simulink model "AlphaBotKreisfahrt"  (R2026b)
settings: Solver=FixedStepDiscrete  StopTime=inf  FixedStep=PAR_Sys_AbtastBasis_f64  EnableMultiTasking=on
StopFcn:
  | SpeichereKreisfahrt('AlphaBotKreisfahrt');
model workspace (MAT data in the model file):
  PAR_AktMot_PWM0_u8 = 80
  PAR_AktMot_RichtL_u8 = 0
  PAR_AktMot_RichtR_u8 = 0
  PAR_AktMot_Start_f32 = Simulink.Parameter
  PAR_AktMot_Start_f32.Value = 0
  PAR_AktMot_Start_f32.Complexity = 'real'
  PAR_AktMot_Start_f32.Dimensions = [1 1]
  PAR_AktMot_Start_f32.DataType = 'single'
  PAR_RegKrs_Ki_f32 = 2
  PAR_RegKrs_Kp_f32 = 0.20000000298
  PAR_RegKrs_RSoll_f32 = 1
  PAR_RegKrs_TKreis_f64 = 40
  PAR_RegKrs_VSoll_f32 = 0.34999999404
  PAR_SenGyr_NKalib_f64 = 1000
  PAR_SenGyr_Vorz_f32 = 1
  PAR_SenOdo_IncU_f32 = 40
  PAR_SenOdo_KorrSL_f32 = 1
  PAR_SenOdo_RadR_f32 = 0.0320000015199
  PAR_SenOdo_Spur_f32 = 0.140000000596
  PAR_Sys_AbtastBasis_f64 = 0.01
  PAR_Sys_Abtast_f64 = 0.01
libraries: arduinolib x8, arduinosensorlib x1
settings Model: SILPILModeSetting=veronly  SimulationMode=external
settings SolverCC: AutoInsertRateTranBlk=on
settings OptimizationCC: DifferentSizesBufferReuse=on  EfficientTunableParamExpr=on  EnhancedBackFolding=on  MaxStackSize=64  OptimizationCustomize=off  OptimizeBlockOrder=speed  PassReuseOutputArgsAs=Individual arguments  RemoveInternalMemoryZeroInit=on  RemoveRootLevelIOMemoryZeroInit=on
settings DebuggingCC: ParameterTunabilityLossMsg=error
settings HardwareCC: ProdHWDeviceType=ARM Compatible->ARM Cortex  ProdLargestAtomicFloat=Double  ProdLargestAtomicInteger=Long
settings SFSimCC: MATLABDynamicMemAlloc=off
settings RTWCC: BuildConfiguration=Faster Runs  Description=Embedded Coder  HardwareBoard=Arduino Uno R4 WiFi  SystemTargetFile=ert.tlc  TLCOptions=-aInlineSetEventsForThisBaseRateFcn=TLC_FALSE -aSuppressMultiTaskScheduler=TLC_FALSE -aRateBasedStepFcn=1  TemplateMakefile=ert_default_tmf  Toolchain=Arduino ARM M4
settings CodeAppCC: ForceParamTrailComments=on  IgnoreCustomStorageClasses=off  InsertBlockDesc=on  OperatorAnnotations=on  SFDataObjDesc=on  SimulinkDataObjDesc=on
settings ERTTargetCC: CombineSignalStateStructs=on  ExtModeAutomaticAllocSize=off  ExtModeIntrfLevel=Level2 - Open  ExtModeMexFile=ext_xcp  ExtModeStaticAlloc=on  SupportContinuousTime=on  SupportVariableSizeSignals=on

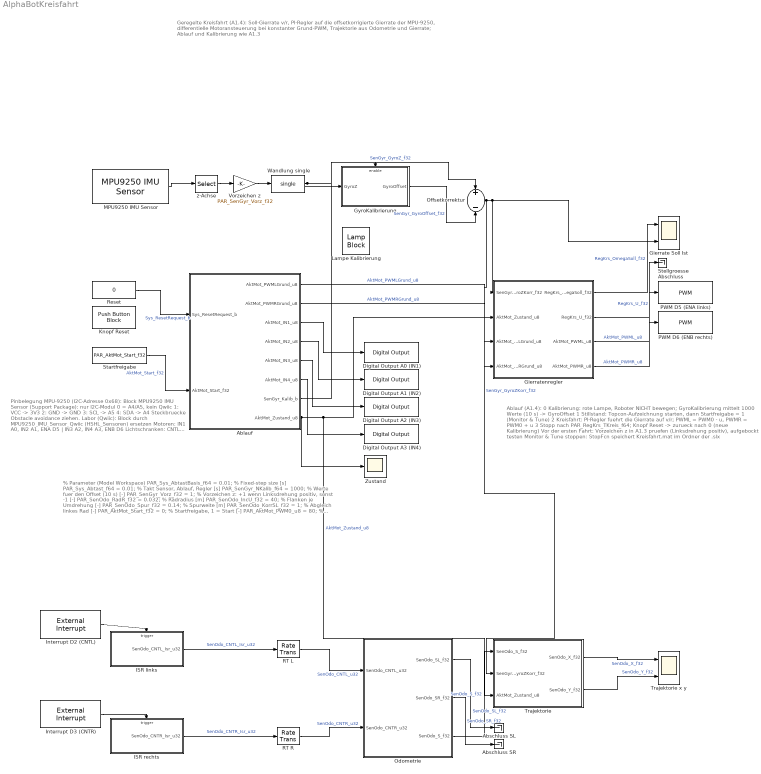
== system AlphaBotKreisfahrt ==
  note: % Parameter (Model Workspace)
      | PAR_Sys_AbtastBasis_f64 = 0.01; % Fixed-step size [s]
      | PAR_Sys_Abtast_f64 = 0.01; % Takt Sensor, Ablauf, Regler [s]
      | PAR_SenGyr_NKalib_f64 = 1000; % Werte fuer den Offset (10 s) [-]
      | PAR_SenGyr_Vorz_f32 = 1; % Vorzeichen z: +1 wenn Linksdrehung positiv, sonst -1 [-]
      | PAR_SenOdo_RadR_f32 = 0.032; % Radradius [m]
      | PAR_SenOdo_IncU_f32 = 40; % Flanken je Umdrehung [-]
      | PAR_SenOdo_Spur_f32 = 0.14; % Spurweite [m]
      | PAR_SenOdo_KorrSL_f32 = 1; % Abgleich linkes Rad [-]
      | PAR_AktMot_Start_f32 = 0; % Startfreigabe, 1 = Start [-]
      | PAR_AktMot_PWM0_u8 = 80; % Grund-PWM, mittlere Geschwindigkeit [-]
      | PAR_AktMot_RichtL_u8 = 0; % IN1 vorwaerts links, IN2 = 1 - IN1 [-]
      | PAR_AktMot_RichtR_u8 = 1; % IN3 vorwaerts rechts, IN4 = 1 - IN3 [-]
      | PAR_RegKrs_VSoll_f32 = 0.35; % Sollgeschwindigkeit [m/s]
      | PAR_RegKrs_RSoll_f32 = 1.0; % Sollradius [m]
      | PAR_RegKrs_Kp_f32 = 0.2; % PI: Verstaerkung [1/(Grad/s)]
      | PAR_RegKrs_Ki_f32 = 2.0; % PI: Integralverstaerkung [1/Grad]
      | PAR_RegKrs_TKreis_f64 = 40; % Dauer Kreisfahrt [s]
  note: Geregelte Kreisfahrt (A1.4): Soll-Gierrate v/r, PI-Regler auf die offsetkorrigierte Gierrate der MPU-9250, differentielle Motoransteuerung bei konstanter Grund-PWM, Trajektorie aus Odometrie und Gierrate; Ablauf und Kalibrierung wie A1.3
  note: Pinbelegung MPU-9250 (I2C-Adresse 0x68):
      | Block MPU9250 IMU Sensor (Support Package): nur I2C-Modul 0 = A4/A5, kein Qwiic
      | 1: VCC -> 3V3 2: GND -> GND 3: SCL -> A5 4: SDA -> A4
      | Steckbruecke Obstacle avoidance ziehen. Labor (Qwiic): Block durch MPU9250_IMU_Sensor_Qwiic (HSHL_Sensoren) ersetzen
      | Motoren: IN1 A0, IN2 A1, ENA D5 | IN3 A2, IN4 A3, ENB D6
      | Lichtschranken: CNTL D2, CNTR D3 (Interrupt, CHANGE)
  note: Ablauf (A1.4):
      | 0 Kalibrierung: rote Lampe, Roboter NICHT bewegen; GyroKalibrierung mittelt 1000 Werte (10 s) -> GyroOffset
      | 1 Stillstand: Topcon-Aufzeichnung starten, dann Startfreigabe = 1 (Monitor & Tune)
      | 2 Kreisfahrt: PI-Regler fuehrt die Gierrate auf v/r; PWML = PWM0 - u, PWMR = PWM0 + u
      | 3 Stopp nach PAR_RegKrs_TKreis_f64; Knopf Reset -> zurueck nach 0 (neue Kalibrierung)
      | Vor der ersten Fahrt: Vorzeichen z in A1.3 pruefen (Linksdrehung positiv), aufgebockt testen
      | Monitor & Tune stoppen: StopFcn speichert Kreisfahrt.mat im Ordner der .slx
  Ablauf : Stateflow chart  TreatAsAtomicUnit=on
  Abschluss SL : Terminator
  Abschluss SR : Terminator
  Digital Output A0 (IN1) : arduinolib/Digital Output  pinNumber=14  Direction=output  blockPlatform=arduino
  Digital Output A1 (IN2) : arduinolib/Digital Output  pinNumber=15  Direction=output  blockPlatform=arduino
  Digital Output A2 (IN3) : arduinolib/Digital Output  pinNumber=16  Direction=output  blockPlatform=arduino
  Digital Output A3 (IN4) : arduinolib/Digital Output  pinNumber=17  Direction=output  blockPlatform=arduino
  Gierrate Soll Ist : Scope  NumInputPorts=2
  Gierratenregler : MATLAB Function  TreatAsAtomicUnit=on
  GyroKalibrierung : Subsystem  TreatAsAtomicUnit=on
  ISR links : Subsystem  TreatAsAtomicUnit=on
  ISR rechts : Subsystem  TreatAsAtomicUnit=on
  Interrupt D2 (CNTL) : arduinolib/External Interrupt  Pin=2  PullUp=off  Mode=CHANGE  InterruptSimulationInput=off
  Interrupt D3 (CNTR) : arduinolib/External Interrupt  Pin=3  PullUp=off  Mode=CHANGE  InterruptSimulationInput=off
  Knopf Reset : PushButtonBlock  ButtonText=Reset  IconOnColor=[0.0, 0.39215686274509803, 0.0]  IconOffColor=[0.0, 1.0, 0.0]
  Lampe Kalibrierung : LampBlock  LabelPosition=Hide  DefaultColor=[192.0, 192.0, 192.0]
  MPU9250 IMU Sensor : arduinosensorlib/MPU9250 IMU Sensor  I2CModule=0  SlaveAddress=0x68  Accel=off  AngularRate=on  Ak8963Field=off  Temperature=off  Status=off  EulerAngles=off  Quat=off  Timestamp=off  AccelRange=2G  Acceldlpf=218.1 Hz  GyroRange=250 dps  Gyrodlpf=41 Hz  DmpOdr=200 Hz  spf=1  SampleTime=PAR_Sys_Abtast_f64  QueueSizeFactor=1
  Odometrie : MATLAB Function  TreatAsAtomicUnit=on
  Offsetkorrektur : Sum  Inputs=+-
  PWM D5 (ENA links) : arduinolib/PWM  pinNumber=5  frequencyType=Default  desiredFrequency=490.2  achievableFrequency=490.2
  PWM D6 (ENB rechts) : arduinolib/PWM  pinNumber=6  frequencyType=Default  desiredFrequency=490.2  achievableFrequency=490.2
  RT L : RateTransition  Deterministic=off  OutPortSampleTime=PAR_Sys_Abtast_f64
  RT R : RateTransition  Deterministic=off  OutPortSampleTime=PAR_Sys_Abtast_f64
  Reset : Constant  Value=0  OutDataTypeStr=boolean  SampleTime=PAR_Sys_Abtast_f64
  Startfreigabe : Constant  Value=PAR_AktMot_Start_f32  OutDataTypeStr=single  SampleTime=PAR_Sys_Abtast_f64
  Stellgroesse Abschluss : Terminator
  Trajektorie : MATLAB Function  TreatAsAtomicUnit=on
  Trajektorie x y : Scope  NumInputPorts=2
  Vorzeichen z : Gain  Gain=PAR_SenGyr_Vorz_f32
  Wandlung single : DataTypeConversion  OutDataTypeStr=single  SaturateOnIntegerOverflow=off  RndMeth=Floor
  Zustand : Scope
  z-Achse : Selector  NumberOfDimensions=2  InputPortWidth=3  IndexOptions=Index vector (dialog),Index vector (dialog)  Indices=3,1  OutputSizes=1
  wires:
  MPU9250 IMU Sensor/1 -> z-Achse/1
  Wandlung single/1 -> GyroKalibrierung/1(GyroZ), Offsetkorrektur/1  "SenGyr_GyroZ_f32"
  GyroKalibrierung/1(GyroOffset) -> Offsetkorrektur/2  "SenGyr_GyroOffset_f32"
  Reset/1 -> Ablauf/1(Sys_ResetRequest_b)  "Sys_ResetRequest_b"
  Startfreigabe/1 -> Ablauf/2(AktMot_Start_f32)  "AktMot_Start_f32"
  Ablauf/3(AktMot_IN1_u8) -> Digital Output A0 (IN1)/1
  Ablauf/4(AktMot_IN2_u8) -> Digital Output A1 (IN2)/1
  Ablauf/5(AktMot_IN3_u8) -> Digital Output A2 (IN3)/1
  Ablauf/6(AktMot_IN4_u8) -> Digital Output A3 (IN4)/1
  Ablauf/7(SenGyr_Kalib_b) -> GyroKalibrierung/Enable
  Ablauf/8(AktMot_Zustand_u8) -> Gierratenregler/2(AktMot_Zustand_u8), Trajektorie/3(AktMot_Zustand_u8), Zustand/1  "AktMot_Zustand_u8"
  z-Achse/1 -> Vorzeichen z/1
  Vorzeichen z/1 -> Wandlung single/1
  Offsetkorrektur/1 -> Gierratenregler/1(SenGyr_GyroZKorr_f32), Gierrate Soll Ist/2, Trajektorie/2(SenGyr_GyroZKorr_f32)  "SenGyr_GyroZKorr_f32"
  Ablauf/1(AktMot_PWMLGrund_u8) -> Gierratenregler/3(AktMot_PWMLGrund_u8)  "AktMot_PWMLGrund_u8"
  Ablauf/2(AktMot_PWMRGrund_u8) -> Gierratenregler/4(AktMot_PWMRGrund_u8)  "AktMot_PWMRGrund_u8"
  Gierratenregler/1(RegKrs_OmegaSoll_f32) -> Gierrate Soll Ist/1  "RegKrs_OmegaSoll_f32"
  Gierratenregler/2(RegKrs_U_f32) -> Stellgroesse Abschluss/1  "RegKrs_U_f32"
  Gierratenregler/3(AktMot_PWML_u8) -> PWM D5 (ENA links)/1  "AktMot_PWML_u8"
  Gierratenregler/4(AktMot_PWMR_u8) -> PWM D6 (ENB rechts)/1  "AktMot_PWMR_u8"
  Interrupt D2 (CNTL)/1 -> ISR links/Trigger
  Interrupt D3 (CNTR)/1 -> ISR rechts/Trigger
  ISR links/1(SenOdo_CNTL_Isr_u32) -> RT L/1  "SenOdo_CNTL_Isr_u32"
  ISR rechts/1(SenOdo_CNTR_Isr_u32) -> RT R/1  "SenOdo_CNTR_Isr_u32"
  RT L/1 -> Odometrie/1(SenOdo_CNTL_u32)  "SenOdo_CNTL_u32"
  RT R/1 -> Odometrie/2(SenOdo_CNTR_u32)  "SenOdo_CNTR_u32"
  Odometrie/1(SenOdo_SL_f32) -> Abschluss SL/1  "SenOdo_SL_f32"
  Odometrie/2(SenOdo_SR_f32) -> Abschluss SR/1  "SenOdo_SR_f32"
  Odometrie/3(SenOdo_S_f32) -> Trajektorie/1(SenOdo_S_f32)  "SenOdo_S_f32"
  Trajektorie/1(SenOdo_X_f32) -> Trajektorie x y/1  "SenOdo_X_f32"
  Trajektorie/2(SenOdo_Y_f32) -> Trajektorie x y/2  "SenOdo_Y_f32"

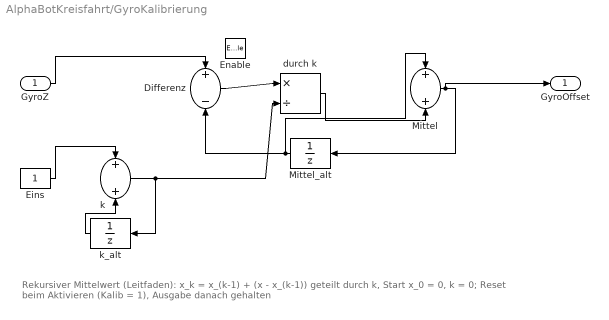
== system AlphaBotKreisfahrt/GyroKalibrierung ==
  note: Rekursiver Mittelwert (Leitfaden): x_k = x_(k-1) + (x - x_(k-1)) geteilt durch k, Start x_0 = 0, k = 0; Reset beim Aktivieren (Kalib = 1), Ausgabe danach gehalten
  GyroZ : Inport
  Enable : EnablePort  StatesWhenEnabling=reset
  Differenz : Sum  Inputs=+-
  Eins : Constant  OutDataTypeStr=single
  Mittel : Sum
  Mittel_alt : UnitDelay  SampleTime=-1
  durch k : Product  Inputs=*/
  k : Sum
  k_alt : UnitDelay  SampleTime=-1
  GyroOffset : Outport  InitialOutput=0
  wires:
  GyroZ/1 -> Differenz/1
  Mittel_alt/1 -> Differenz/2, Mittel/1
  Differenz/1 -> durch k/1
  Eins/1 -> k/1
  k_alt/1 -> k/2
  k/1 -> k_alt/1, durch k/2
  durch k/1 -> Mittel/2
  Mittel/1 -> Mittel_alt/1, GyroOffset/1

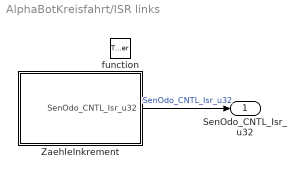
== system AlphaBotKreisfahrt/ISR links ==
  function : TriggerPort  TriggerType=function-call  VariantControl=(inherit)
  ZaehleInkrement : MATLAB Function  TreatAsAtomicUnit=on
  SenOdo_CNTL_Isr_u32 : Outport
  wires:
  ZaehleInkrement/1(SenOdo_CNTL_Isr_u32) -> SenOdo_CNTL_Isr_u32/1  "SenOdo_CNTL_Isr_u32"

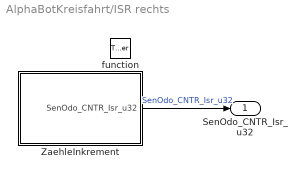
== system AlphaBotKreisfahrt/ISR rechts ==
  function : TriggerPort  TriggerType=function-call  VariantControl=(inherit)
  ZaehleInkrement : MATLAB Function  TreatAsAtomicUnit=on
  SenOdo_CNTR_Isr_u32 : Outport
  wires:
  ZaehleInkrement/1(SenOdo_CNTR_Isr_u32) -> SenOdo_CNTR_Isr_u32/1  "SenOdo_CNTR_Isr_u32"

== matlab function AlphaBotKreisfahrt/Trajektorie ==
  data: SenOdo_S_f32 input single; SenOdo_X_f32 output; SenGyr_GyroZKorr_f32 input single; AktMot_Zustand_u8 input uint8; SenOdo_Y_f32 output; PAR_Sys_Abtast_f64 parameter
function [SenOdo_X_f32,SenOdo_Y_f32] = BerechneTrajektorie(SenOdo_S_f32,SenGyr_GyroZKorr_f32,AktMot_Zustand_u8,PAR_Sys_Abtast_f64)
% BerechneTrajektorie: Position aus Odometrie-Strecke und Gierrate (A1.4, D5)
% Eingabe:  SenOdo_S_f32 [1x1]: mittlere Strecke (SL + SR)/2 [m]
%           SenGyr_GyroZKorr_f32 [1x1]: offsetkorrigierte Gierrate [Grad/s]
%           AktMot_Zustand_u8 [1x1]: Zustand des Ablaufs [-], PAR_Sys_Abtast_f64 Abtastzeit [s]
% Ausgabe:  SenOdo_X_f32, SenOdo_Y_f32 [1x1]: Position, Ursprung und Richtung x beim Start der Kreisfahrt [m]
persistent fX fY fPsi fSAlt   % Position [m], Kurs [rad], Strecke im vorigen Schritt [m]

if isempty(fX)
    fX = single(0);
    fY = single(0);
    fPsi = single(0);
    fSAlt = SenOdo_S_f32;
end
fDeltaS = SenOdo_S_f32 - fSAlt;   % Weg im Takt [m]
fSAlt = SenOdo_S_f32;
% Kurs aus der Gierrate, Weg aus der Odometrie, Mittelpunktregel; vor der Kreisfahrt Ursprung
if AktMot_Zustand_u8 < 2
    fX = single(0);
    fY = single(0);
    fPsi = single(0);
else
    fDeltaPsi = SenGyr_GyroZKorr_f32 * single(pi / 180) * single(PAR_Sys_Abtast_f64);   % Kursaenderung [rad]
    fX = fX + fDeltaS * cos(fPsi + fDeltaPsi / 2);
    fY = fY + fDeltaS * sin(fPsi + fDeltaPsi / 2);
    fPsi = fPsi + fDeltaPsi;
end
SenOdo_X_f32 = fX;
SenOdo_Y_f32 = fY;
end

== matlab function AlphaBotKreisfahrt/ISR links/ZaehleInkrement ==
  data: SenOdo_CNTL_Isr_u32 output
function SenOdo_CNTL_Isr_u32 = ZaehleInkrement()
% ZaehleInkrement: ISR je Flanke der Lichtschranke (Modus CHANGE)
% Ausgabe:  SenOdo_CNTL_Isr_u32 [1x1]: Flanken seit Programmstart [-]
persistent nZaehler   % Flankenzaehler [-]

if isempty(nZaehler)
    nZaehler = uint32(0);
end
nZaehler = nZaehler + 1;
SenOdo_CNTL_Isr_u32 = nZaehler;
end

== matlab function AlphaBotKreisfahrt/Gierratenregler ==
  data: SenGyr_GyroZKorr_f32 input single; RegKrs_OmegaSoll_f32 output; AktMot_Zustand_u8 input uint8; AktMot_PWMLGrund_u8 input uint8; AktMot_PWMRGrund_u8 input uint8; RegKrs_U_f32 output; AktMot_PWML_u8 output; AktMot_PWMR_u8 output; PAR_RegKrs_VSoll_f32 parameter; PAR_RegKrs_RSoll_f32 parameter; PAR_RegKrs_Kp_f32 parameter; PAR_RegKrs_Ki_f32 parameter; PAR_Sys_Abtast_f64 parameter
function [RegKrs_OmegaSoll_f32,RegKrs_U_f32,AktMot_PWML_u8,AktMot_PWMR_u8] = RegleGierrate(SenGyr_GyroZKorr_f32,AktMot_Zustand_u8,AktMot_PWMLGrund_u8,AktMot_PWMRGrund_u8,PAR_RegKrs_VSoll_f32, PAR_RegKrs_RSoll_f32, PAR_RegKrs_Kp_f32, PAR_RegKrs_Ki_f32, PAR_Sys_Abtast_f64)
% RegleGierrate: PI-Regler der Gierrate fuer die Kreisfahrt (A1.4)
% Eingabe:  SenGyr_GyroZKorr_f32 [1x1]: offsetkorrigierte Gierrate [Grad/s]
%           AktMot_Zustand_u8 [1x1]: 0 Kalibrierung, 1 Stillstand, 2 Kreisfahrt, 3 Stopp [-]
%           AktMot_PWMLGrund_u8, AktMot_PWMRGrund_u8 [1x1]: PWM0 in Kreisfahrt, sonst 0 [-]
%           PAR_RegKrs_VSoll_f32 Sollgeschwindigkeit [m/s], PAR_RegKrs_RSoll_f32 Sollradius [m]
%           PAR_RegKrs_Kp_f32 [1/(Grad/s)], PAR_RegKrs_Ki_f32 [1/Grad], PAR_Sys_Abtast_f64 [s]
% Ausgabe:  RegKrs_OmegaSoll_f32 [1x1]: Soll-Gierrate v/r [Grad/s]
%           RegKrs_U_f32 [1x1]: Stellgroesse u = KP*e + KI*Summe(e*T), |u| <= PWM0 [-]
%           AktMot_PWML_u8, AktMot_PWMR_u8 [1x1]: PWM0 - u, PWM0 + u, begrenzt auf 0...255 [-]
persistent fIntegral   % I-Anteil [-]

if isempty(fIntegral)
    fIntegral = single(0);
end
% D1: omega_soll = v / r in Grad/s
RegKrs_OmegaSoll_f32 = PAR_RegKrs_VSoll_f32 / PAR_RegKrs_RSoll_f32 * single(180 / pi);
fFehler = RegKrs_OmegaSoll_f32 - SenGyr_GyroZKorr_f32;   % Regelfehler e [Grad/s]
fUMax = single(AktMot_PWMLGrund_u8);   % Stellbereich |u| <= PWM0 [-]
% D3: PI nur in Kreisfahrt; an der Stellgrenze wird nicht weiter integriert (Anti-Windup)
RegKrs_U_f32 = single(0);
if AktMot_Zustand_u8 == 2
    fIntNeu = fIntegral + PAR_RegKrs_Ki_f32 * fFehler * single(PAR_Sys_Abtast_f64);   % I-Anteil neu [-]
    RegKrs_U_f32 = PAR_RegKrs_Kp_f32 * fFehler + fIntNeu;
    if abs(RegKrs_U_f32) <= fUMax
        fIntegral = fIntNeu;
    else
        RegKrs_U_f32 = min(max(RegKrs_U_f32,-fUMax),fUMax);
    end
else
    fIntegral = single(0);
end
% D4: differentielle Ansteuerung; u > 0 dreht nach links (Gierrate positiv)
AktMot_PWML_u8 = uint8(single(AktMot_PWMLGrund_u8) - RegKrs_U_f32);
AktMot_PWMR_u8 = uint8(single(AktMot_PWMRGrund_u8) + RegKrs_U_f32);
end

== stateflow chart AlphaBotKreisfahrt/Ablauf ==
  settings: updateMethod=DISCRETE  sampleTime=PAR_Sys_Abtast_f64
  state Kalibrierung
    entry:
    AktMot_PWMLGrund_u8 = uint8(0);
    AktMot_PWMRGrund_u8 = uint8(0);
    AktMot_IN1_u8 = uint8(0);
    AktMot_IN2_u8 = uint8(0);
    AktMot_IN3_u8 = uint8(0);
    AktMot_IN4_u8 = uint8(0);
    SenGyr_Kalib_b = true;
    AktMot_Zustand_u8 = uint8(0);
    during:
    SenGyr_Kalib_b = ~Sys_ResetRequest_b;
    Kalibrierung -> Kalibrierung [order 1] : [Sys_ResetRequest_b]
  state Stillstand
    entry:
    AktMot_PWMLGrund_u8 = uint8(0);
    AktMot_PWMRGrund_u8 = uint8(0);
    AktMot_IN1_u8 = uint8(0);
    AktMot_IN2_u8 = uint8(0);
    AktMot_IN3_u8 = uint8(0);
    AktMot_IN4_u8 = uint8(0);
    SenGyr_Kalib_b = false;
    AktMot_Zustand_u8 = uint8(1);
  state Kreisfahrt
    entry:
    AktMot_PWMLGrund_u8 = PAR_AktMot_PWM0_u8;
    AktMot_PWMRGrund_u8 = PAR_AktMot_PWM0_u8;
    AktMot_IN1_u8 = PAR_AktMot_RichtL_u8;
    AktMot_IN2_u8 = uint8(1) - PAR_AktMot_RichtL_u8;
    AktMot_IN3_u8 = PAR_AktMot_RichtR_u8;
    AktMot_IN4_u8 = uint8(1) - PAR_AktMot_RichtR_u8;
    SenGyr_Kalib_b = false;
    AktMot_Zustand_u8 = uint8(2);
  state Stopp
    entry:
    AktMot_PWMLGrund_u8 = uint8(0);
    AktMot_PWMRGrund_u8 = uint8(0);
    AktMot_IN1_u8 = uint8(0);
    AktMot_IN2_u8 = uint8(0);
    AktMot_IN3_u8 = uint8(0);
    AktMot_IN4_u8 = uint8(0);
    SenGyr_Kalib_b = false;
    AktMot_Zustand_u8 = uint8(3);
  (default) -> Kalibrierung
  Stillstand -> Kalibrierung [order 1] : [Sys_ResetRequest_b]
  Kalibrierung -> Stillstand [order 1] : [after(PAR_SenGyr_NKalib_f64,tick)]
  Kreisfahrt -> Kalibrierung [order 1] : [Sys_ResetRequest_b]
  Stillstand -> Kreisfahrt [order 2] : [AktMot_Start_f32 >= 1]
  Stopp -> Kalibrierung : [Sys_ResetRequest_b]
  Kreisfahrt -> Stopp [order 2] : [after(PAR_RegKrs_TKreis_f64,sec)]
  data: Sys_ResetRequest_b input boolean; AktMot_Start_f32 input single; AktMot_PWMLGrund_u8 output uint8; AktMot_PWMRGrund_u8 output uint8; AktMot_IN1_u8 output uint8; AktMot_IN2_u8 output uint8; AktMot_IN3_u8 output uint8; AktMot_IN4_u8 output uint8; SenGyr_Kalib_b output boolean; AktMot_Zustand_u8 output uint8; PAR_SenGyr_NKalib_f64 parameter; PAR_RegKrs_TKreis_f64 parameter; PAR_AktMot_RichtL_u8 parameter; PAR_AktMot_RichtR_u8 parameter; PAR_AktMot_PWM0_u8 parameter

== matlab function AlphaBotKreisfahrt/ISR rechts/ZaehleInkrement ==
  data: SenOdo_CNTR_Isr_u32 output
function SenOdo_CNTR_Isr_u32 = ZaehleInkrement()
% ZaehleInkrement: ISR je Flanke der Lichtschranke (Modus CHANGE)
% Ausgabe:  SenOdo_CNTR_Isr_u32 [1x1]: Flanken seit Programmstart [-]
persistent nZaehler   % Flankenzaehler [-]

if isempty(nZaehler)
    nZaehler = uint32(0);
end
nZaehler = nZaehler + 1;
SenOdo_CNTR_Isr_u32 = nZaehler;
end

== matlab function AlphaBotKreisfahrt/Odometrie ==
  settings: updateMethod=DISCRETE  sampleTime=PAR_Sys_Abtast_f64
  data: SenOdo_CNTL_u32 input; SenOdo_SL_f32 output; SenOdo_CNTR_u32 input; SenOdo_SR_f32 output; SenOdo_S_f32 output; PAR_SenOdo_RadR_f32 parameter; PAR_SenOdo_IncU_f32 parameter; PAR_SenOdo_KorrSL_f32 parameter
function [SenOdo_SL_f32,SenOdo_SR_f32,SenOdo_S_f32] = BerechneStrecke(SenOdo_CNTL_u32,SenOdo_CNTR_u32,PAR_SenOdo_RadR_f32,PAR_SenOdo_IncU_f32,PAR_SenOdo_KorrSL_f32)
% BerechneStrecke: Radstrecken und mittlere Strecke aus den Flankenzaehlern
% Eingabe:  SenOdo_CNTL_u32, SenOdo_CNTR_u32 [1x1]: Flanken links, rechts [-]
%           PAR_SenOdo_RadR_f32 Radradius [m], PAR_SenOdo_IncU_f32 Flanken je Umdrehung [-]
%           PAR_SenOdo_KorrSL_f32 Abgleichfaktor linkes Rad, Start 1 [-]
% Ausgabe:  SenOdo_SL_f32, SenOdo_SR_f32 [1x1]: Radstrecke links, rechts [m]
%           SenOdo_S_f32                 [1x1]: mittlere Strecke s = (sL + sR)/2 [m]
fWegInkrement = 2 * single(pi) * PAR_SenOdo_RadR_f32 / PAR_SenOdo_IncU_f32;   % Weg je Flanke [m]
SenOdo_SL_f32 = single(SenOdo_CNTL_u32) * fWegInkrement * PAR_SenOdo_KorrSL_f32;
SenOdo_SR_f32 = single(SenOdo_CNTR_u32) * fWegInkrement;
SenOdo_S_f32 = (SenOdo_SL_f32 + SenOdo_SR_f32) / 2;
end
